simulink model "ECO_RM_WEC_DDLG_PI"  (R2025a)
settings: Solver=ode4  StartTime=0  StopTime=120  FixedStep=0.00025  MaxStep=0.00025  RelTol=1e-3
values from neighbouring files (symbols this model uses):
  Ki_DDLG = alpha*Kp_DDLG    [DDLG_PI_compensated_analysis.m]    (also in wecSimInputFile.m = 4993.87518575)
  Kp_DDLG = rho/abs(Lshape0)    [DDLG_PI_compensated_analysis.m]    (also in wecSimInputFile.m = 1625.0963416)
undefined symbols (not defined in the file or in its folder): body, constraint, geometry, hydroData, pto, ptoSim
libraries: WECSim_Lib_Body_Elements x2, WECSim_Lib_PTOSim x1, WECSim_Lib_Frames x1, slpidlib x1, WECSim_Lib_Constraints x1, WECSim_Lib_PTOs x1
settings Model: Creator=pam1061  LastModifiedBy=Viki Vagnerova
settings SolverCC: ZeroCrossControl=DisableAll  AutoInsertRateTranBlk=on
settings DataIOCC: ReturnWorkspaceOutputs=off
settings OptimizationCC: SimCompilerOptimization=on

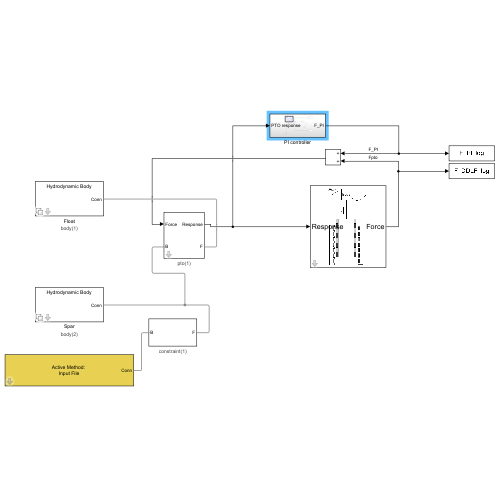
[thumbnail: Simulink's stored preview of the top-level diagram]
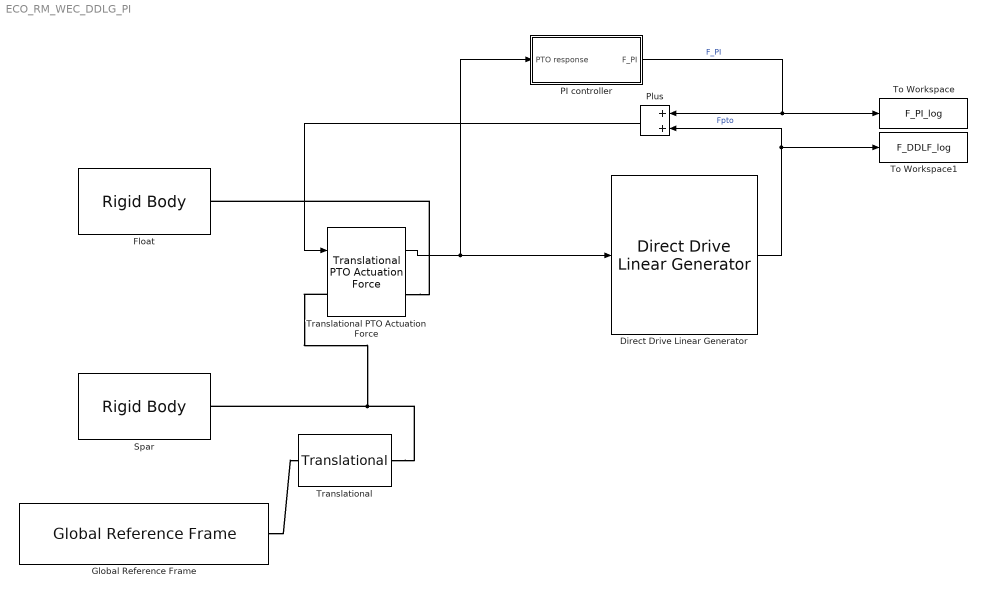
== system ECO_RM_WEC_DDLG_PI ==
  Direct Drive Linear Generator : WECSim_Lib_PTOSim/Electric/Direct Drive Linear Generator  ptoSim=ptoSim(1)  Rs=0  Ls=0  Rload=0  Bfric=0  tau_p=0  theta_d_0=0  lambda_sd_0=0  lambda_sq_0=0  lambda_fd=0
  Float : WECSim_Lib_Body_Elements/Rigid Body  body=body(1)  h5File=hydroData/*.h5  geometryFile=geometry/*.stl  mass=0  inertia=0 0 0  inertiaProducts=0 0 0  nonHydro=0  nonlinearHydro=0  centerGravity=0 0 0  centerBuoyancy=0 0 0  dof=6  volume=0  displacement=0 0 0  axis=0 1 0  angle=0  option=0  cd=0 0 0  ca=0 0 0  area=0 0 0  VME=0  rgME=0 0 0  z=0 0 1
  Global Reference Frame : WECSim_Lib_Frames/Global Reference Frame  waves=waves  simu=simu  InputMethod=Input File  InputFile=wecSimInputFile.m  mode=normal  explorer=off  solver=ode4  startTime=0  rampTime=100  endTime=400  dt=0.1  cicEndTime=60  stateSpace=0  WaveClass=regular  height=2.5  period=8  elevationFile=NOT DEFINED  spectrumFile=NOT DEFINED  direction=0  spread=1  spectrumType=NOT DEFINED  phaseSeed=0  option=EqualEnergy
  PI controller : Subsystem
  Plus : Sum
  Spar : WECSim_Lib_Body_Elements/Rigid Body  body=body(2)  h5File=hydroData/*.h5  geometryFile=geometry/*.stl  mass=0  inertia=0 0 0  inertiaProducts=0 0 0  nonHydro=0  nonlinearHydro=0  centerGravity=0 0 0  centerBuoyancy=0 0 0  dof=6  volume=0  displacement=0 0 0  axis=0 1 0  angle=0  option=0  cd=0 0 0  ca=0 0 0  area=0 0 0  VME=0  rgME=0 0 0  z=0 0 1
  To Workspace : ToWorkspace  VariableName=F_PI_log  SaveFormat=Timeseries  SampleTime=-1
  To Workspace1 : ToWorkspace  VariableName=F_DDLF_log  SaveFormat=Timeseries  SampleTime=-1
  Translational : WECSim_Lib_Constraints/Translational  constraint=constraint(1)  loc="0  0  0"  displacement=0 0 0  y=0 1 0  z=0 0 1  upperLimitSpecify=off  upperLimitBound=0  upperLimitTransitionRegionWidth=0  upperLimitStiffness=0  upperLimitDamping=0  lowerLimitSpecify=off  lowerLimitBound=0  lowerLimitTransitionRegionWidth=0  lowerLimitStiffness=0  lowerLimitDamping=0
      settings: AttributesFormatString=%<constraint>
  Translational PTO Actuation Force : WECSim_Lib_PTOs/Translational PTO Actuation Force  pto=pto(1)  loc="0  0  0"  stiffness=0  damping=0  equilibriumPosition=0  pretension=0  displacement=0 0 0  y=0 1 0  z=0 0 1  upperLimitSpecify=off  upperLimitBound=0  upperLimitTransitionRegionWidth=0  upperLimitStiffness=0  upperLimitDamping=0  lowerLimitSpecify=off  lowerLimitBound=0  lowerLimitTransitionRegionWidth=0  lowerLimitStiffness=0  lowerLimitDamping=0
      settings: AttributesFormatString=%<pto>
  wires:
  Translational PTO Actuation Force/1 -> PI controller/1(PTO response), Direct Drive Linear Generator/1
  Direct Drive Linear Generator/1 -> Plus/2, To Workspace1/1  "Fpto"
  Plus/1 -> Translational PTO Actuation Force/1
  PI controller/1(F_PI) -> To Workspace/1, Plus/1  "F_PI"
  connections:
  Global Reference Frame/RConn1 -- Translational/LConn1
  Translational/RConn1 -- Translational PTO Actuation Force/LConn1 -- Spar/RConn1
  Translational PTO Actuation Force/RConn1 -- Float/RConn1

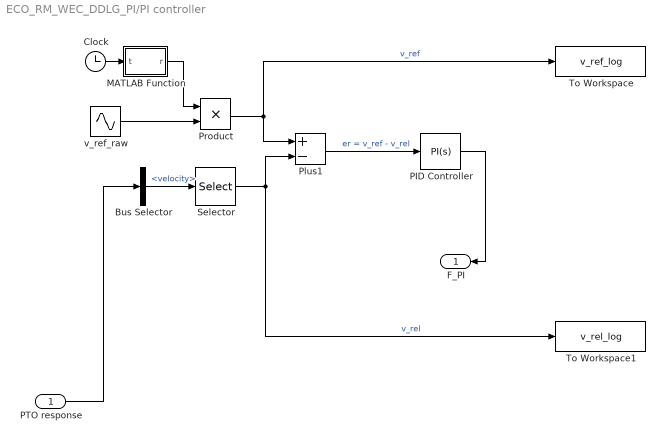
== system ECO_RM_WEC_DDLG_PI/PI controller ==
  PTO response : Inport
  Bus Selector : BusSelector  OutputSignals=velocity
  Clock : Clock
  MATLAB Function : MATLAB Function  TreatAsAtomicUnit=on
  PID Controller : slpidlib/PID Controller  Controller=PI  Form=Parallel  TimeDomain=Continuous-time  UseExternalTs=off  SampleTime=-1  IntegratorMethod=Forward Euler  FilterMethod=Forward Euler  ControllerParametersSource=internal  P=Kp_DDLG  I=Ki_DDLG  UseKiTs=off  D=0  UseExternalDerivativeSource=off  N=100  UseFilter=on  TunerSelectOption=Transfer Function Based (PID Tuner App)  InitialConditionSource=internal  InitialConditionForIntegrator=0  InitialConditionForFilter=0  DifferentiatorICPrevScaledInput=0  ExternalReset=none  TrackingMode=off  Kt=1  LimitOutput=off  SatLimitsSource=internal  UpperSaturationLimit=inf  LowerSaturationLimit=-inf  LinearizeAsGain=on  AntiWindupMode=none  Kb=1  LimitIntegrator=off  UpperIntegratorSaturationLimit=inf  LowerIntegratorSaturationLimit=-inf  POutMin=[]  POutMax=[]  IOutMin=[]  IOutMax=[]  DOutMin=[]  DOutMax=[]  NOutMin=[]  NOutMax=[]  SumOutMin=[]  SumOutMax=[]  SaturationOutMin=[]  SaturationOutMax=[]  PParamMin=[]  PParamMax=[]  IParamMin=[]  IParamMax=[]  DParamMin=[]  DParamMax=[]  NParamMin=[]  NParamMax=[]  KbParamMin=[]  KbParamMax=[]  KtParamMin=[]  KtParamMax=[]  KbOutMin=[]  KbOutMax=[]  KtOutMin=[]  KtOutMax=[]  IntegratorOutMin=[]  IntegratorOutMax=[]  FilterOutMin=[]  FilterOutMax=[]  SumI1OutMin=[]  SumI1OutMax=[]  SumI2OutMin=[]  SumI2OutMax=[]  SumI3OutMin=[]  SumI3OutMax=[]  SumI4OutMin=[]  SumI4OutMax=[]  SumDOutMin=[]  SumDOutMax=[]  DifferentiatorOutMin=[]  DifferentiatorOutMax=[]  FilterDiffOutCoefMin=[]  FilterDiffOutCoefMax=[]  ReciprocalOutMin=[]  ReciprocalOutMax=[]  SumDenOutMin=[]  SumDenOutMax=[]  SumNumOutMin=[]  SumNumOutMax=[]  DivideOutMin=[]  DivideOutMax=[]  UdiffTsProdOutMin=[]  UdiffTsProdOutMax=[]  NTsProdOutMin=[]  NTsProdOutMax=[]  UintegralTsProdOutMin=[]  UintegralTsProdOutMax=[]  UngainTsProdOutMin=[]  UngainTsProdOutMax=[]  ClampingZeroOutDataTypeStr=Inherit: Inherit via back propagation  ClampingZeroOutMin=[]  ClampingZeroOutMax=[]  FilterDenConstantOutDataTypeStr=Inherit: Inherit via back propagation  FilterDenConstantOutMin=[]  FilterDenConstantOutMax=[]  PCopyOutDataTypeStr=Inherit: Inherit via back propagation  PCopyOutMin=[]  PCopyOutMax=[]  NCopyOutDataTypeStr=Inherit: Inherit via back propagation  NCopyOutMin=[]  NCopyOutMax=[]  IntegratorContinuousStateAttributes=''  IntegratorStateMustResolveToSignalObject=off  IntegratorRTWStateStorageClass=Auto  FilterContinuousStateAttributes=''  FilterStateMustResolveToSignalObject=off  FilterRTWStateStorageClass=Auto  ParallelPVariant=InternalParameters  IdealPVariant=Disabled  IVariant=InternalParameters  DVariant=Disabled  IntegratorVariant=Continuous  SatVariant=Disabled  AWVariant=Passthrough  PCopyVariant=Disabled  TRVariant=Disabled  FdbkBlocksVariant=Forward  IdealPFdbkVariant=Disabled  SatFdbkVariant=Disabled  DerivativeFilterVariant=Disabled  NVariant=Disabled  NCopyVariant=Disabled_SignalSpec  FilterICVariant=Disabled  IntegratorICVariant=InternalICs  ExternalResetVariant=Disabled  TRSumVariant=Passthrough  SumFdbkVariant=Disabled  SumVariant=Sum_PI  TsampFilterVariant=InternalTs  TsampNgainVariant=Passthrough  TsampIntegralVariant=Disabled_SignalSpec  ExternalSaturationOutDataTypeStr=Inherit: Same as second input  DerivativeSourceVariant=Disabled  PreIntVariant=InternalPreInt
  Plus1 : Sum  Inputs=+-
  Product : Product
  Selector : Selector  InputPortWidth=6  IndexOptions=Index vector (dialog)  Indices=[3]  OutputSizes=1
  To Workspace : ToWorkspace  VariableName=v_ref_log  SaveFormat=Timeseries  SampleTime=-1
  To Workspace1 : ToWorkspace  VariableName=v_rel_log  SaveFormat=Timeseries  SampleTime=-1
  v_ref_raw : Sin  Amplitude=1.039494  Frequency=4  Phase=1.94184  SampleTime=0
  F_PI : Outport
  wires:
  MATLAB Function/1(r) -> Product/1
  v_ref_raw/1 -> Product/2
  PID Controller/1 -> F_PI/1
  Plus1/1 -> PID Controller/1  "er = v_ref - v_rel"
  Selector/1 -> To Workspace1/1, Plus1/2  "v_rel"
  Bus Selector/1 -> Selector/1  "<velocity>"
  Product/1 -> Plus1/1, To Workspace/1  "v_ref"
  Clock/1 -> MATLAB Function/1(t)
  PTO response/1 -> Bus Selector/1

== matlab function ECO_RM_WEC_DDLG_PI/PI controller/MATLAB Function ==
  data: t input; r output
function r = wecRamp(t)

Tr = 30;

if t < Tr
    r = 0.5*(1 - cos(pi*t/Tr));
else
    r = 1;
end
